simulink model "ArmsSimulation"  (R2020b)
settings: Solver=VariableStepAuto  StartTime=0.0  StopTime=10  RelTol=1e-3
settings Model: Creator=Erfan  LastModifiedBy=Erfan

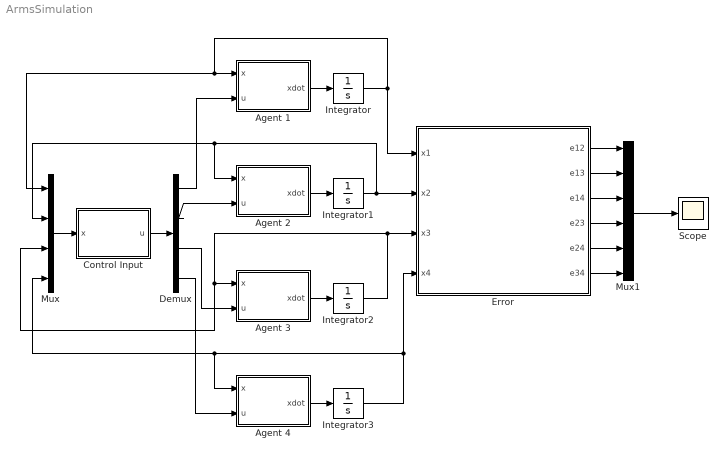
== system ArmsSimulation ==
  Agent 1 : MATLAB Function  TreatAsAtomicUnit=on
  Agent 2 : MATLAB Function  TreatAsAtomicUnit=on
  Agent 3 : MATLAB Function  TreatAsAtomicUnit=on
  Agent 4 : MATLAB Function  TreatAsAtomicUnit=on
  Control Input : MATLAB Function  TreatAsAtomicUnit=on
  Demux : Demux
  Error : MATLAB Function  TreatAsAtomicUnit=on
  Integrator : Integrator  InitialCondition=[1 2]
  Integrator1 : Integrator  InitialCondition=[-1 0]
  Integrator2 : Integrator  InitialCondition=[3 1]
  Integrator3 : Integrator  InitialCondition=[1 -3]
  Mux : Mux
  Mux1 : Mux  Inputs=6
  Scope : Scope
  wires:
  Agent 1/1(xdot) -> Integrator/1
  Integrator/1 -> Error/1(x1), Mux/1, Agent 1/1(x)
  Integrator1/1 -> Error/2(x2), Agent 2/1(x), Mux/2
  Agent 2/1(xdot) -> Integrator1/1
  Agent 3/1(xdot) -> Integrator2/1
  Integrator2/1 -> Mux/3, Agent 3/1(x), Error/3(x3)
  Integrator3/1 -> Agent 4/1(x), Mux/4, Error/4(x4)
  Agent 4/1(xdot) -> Integrator3/1
  Control Input/1(u) -> Demux/1
  Demux/1 -> Agent 1/2(u)
  Demux/2 -> Agent 2/2(u)
  Demux/3 -> Agent 3/2(u)
  Demux/4 -> Agent 4/2(u)
  Mux/1 -> Control Input/1(x)
  Error/1(e12) -> Mux1/1
  Error/2(e13) -> Mux1/2
  Error/3(e14) -> Mux1/3
  Error/4(e23) -> Mux1/4
  Error/5(e24) -> Mux1/5
  Error/6(e34) -> Mux1/6
  Mux1/1 -> Scope/1

== matlab function ArmsSimulation/Agent 2 ==
  data: x input; u input; xdot output
function xdot = fcn(x,u)

J = 0.03;
B = 0.1;
kt = 0.5;

A = [0 1;
    0 -B/J];
B = [0;
    kt/J];

xdot = A*x + B*u;

== matlab function ArmsSimulation/Agent 1 ==
  data: x input; u input; xdot output
function xdot = fcn(x,u)

J = 0.03;
B = 0.1;
kt = 0.5;

A = [0 1;
    0 -B/J];
B = [0;
    kt/J];

xdot = A*x + B*u;

== matlab function ArmsSimulation/Agent 3 ==
  data: x input; u input; xdot output
function xdot = fcn(x,u)

J = 0.03;
B = 0.1;
kt = 0.5;

A = [0 1;
    0 -B/J];
B = [0;
    kt/J];

xdot = A*x + B*u;

== matlab function ArmsSimulation/Agent 4 ==
  data: x input; u input; xdot output
function xdot = fcn(x,u)

J = 0.03;
B = 0.1;
kt = 0.5;

A = [0 1;
    0 -B/J];
B = [0;
    kt/J];

xdot = A*x + B*u;

== matlab function ArmsSimulation/Control Input ==
  data: x input; u output
function u = fcn(x)

K1 = [-0.5525 -0.2164];
K2 = [-0.5525 -0.2164];
K3 = [-0.5525 -0.2164];
K4 = [0 0];

KD = [K1 0 0 0 0 0 0;
    0 0 K2 0 0 0 0;
    0 0 0 0 K3 0 0;
    0 0 0 0 0 0 K4];

LC = [1 0 0 0 0 0 -1 0;
    0 1 0 0 0 0 0 -1;
    0 0 1 0 0 0 -1 0;
    0 0 0 1 0 0 0 -1;
    0 0 0 0 1 0 -1 0;
    0 0 0 0 0 1 0 -1;
    0 0 0 0 0 0 0 0;
    0 0 0 0 0 0 0 0];

u = KD*LC*x;

== matlab function ArmsSimulation/Error ==
  data: x1 input; e12 output; x2 input; x3 input; x4 input; e13 output; e14 output; e23 output; e24 output; e34 output
function [e12,e13,e14,e23,e24,e34] = fcn(x1,x2,x3,x4)

e12 = x1 - x2;
e13 = x1 - x3;
e14 = x1 - x4;
e23 = x2 - x3;
e24 = x2 - x4;
e34 = x3 - x4;
